simulink model "machine_model_A_test"  (R2018b)
settings: Solver=ode45  StartTime=0.0  StopTime=65  RelTol=1e-3
PreLoadFcn:
  | load_system('../simulink_reference_models/test_sequence_lib');
InitFcn:
  | close all
  | clear all
  | 
  | T_CNTL = 1/5e3;
  | 
  | P_NOM = 1e6;
  | VLL_NOM = 480;
  | F_NOM = 60;
  | W_NOM = 2 * 3.14159265 * F_NOM;
  | 
  | Z_BASE = VLL_NOM * VLL_NOM / P_NOM;
  | L_BASE = Z_BASE / W_NOM;
  | C_BASE = 1 / (W_NOM * Z_BASE);
libraries: simulink x4, test_sequence_lib x4
settings Model: SimulationMode=rapid-accelerator  Creator=HussamAlatrash  LastModifiedBy=ahhei
settings DataIOCC: ReturnWorkspaceOutputs=on
settings DebuggingCC: UnconnectedInputMsg=none  UnconnectedOutputMsg=none  UnconnectedLineMsg=none
settings ModelReferenceCC: EnableRefExpFcnMdlSchedulingChecks=off
settings RTWCC: Description=Generic Real-Time Target
settings ConfigComp: CovBoundaryAbsTol=1.0e-5

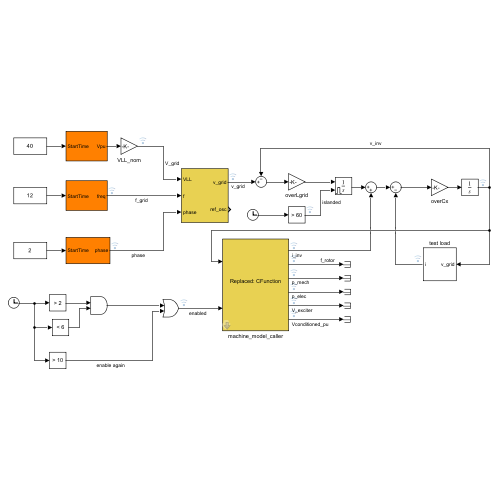
[thumbnail: Simulink's stored preview of the top-level diagram]
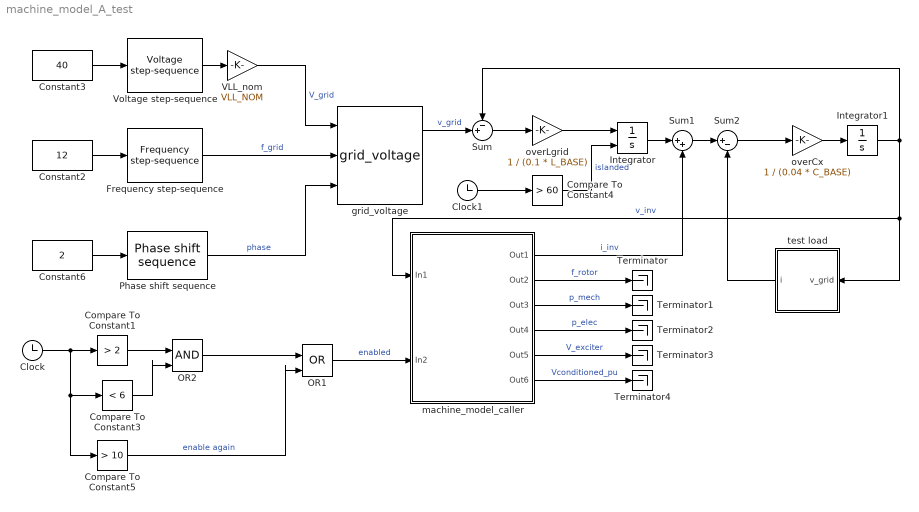
== system machine_model_A_test ==
  Clock : Clock
  Clock1 : Clock
  Compare To Constant1 : simulink/Logic and Bit Operations/Compare To Constant  relop=>  const=2  OutDataTypeStr=boolean
  Compare To Constant3 : simulink/Logic and Bit Operations/Compare To Constant  relop=<  const=6  OutDataTypeStr=boolean
  Compare To Constant4 : simulink/Logic and Bit Operations/Compare To Constant  relop=>  const=60  OutDataTypeStr=boolean
  Compare To Constant5 : simulink/Logic and Bit Operations/Compare To Constant  relop=>  const=10  OutDataTypeStr=boolean
  Constant2 : Constant  Value=12
  Constant3 : Constant  Value=40
  Constant6 : Constant  Value=2
  Frequency step-sequence : test_sequence_lib/Frequency step-sequence  SystemSampleTime=-1  EmptyChoice=off  PassThrough=off  PassThroughVariantControl=(default)  EmptyChoiceVariantControl=(default)  Latency=0  AutoFrameSizeCalculation=off
  Integrator : Integrator  ExternalReset=level
  Integrator1 : Integrator
  OR1 : Logic  Operator=OR  IconShape=distinctive  AllPortsSameDT=off  OutDataTypeStr=boolean
  OR2 : Logic  IconShape=distinctive  AllPortsSameDT=off  OutDataTypeStr=boolean
  Phase shift sequence : test_sequence_lib/Phase shift sequence  SystemSampleTime=-1  EmptyChoice=off  PassThrough=off  PassThroughVariantControl=(default)  EmptyChoiceVariantControl=(default)  Latency=0  AutoFrameSizeCalculation=off
  Sum : Sum  Inputs=-+|
  Sum1 : Sum  Inputs=|++
  Sum2 : Sum  Inputs=|+-
  Terminator{,1..4} (5 alike) : Terminator
  VLL_nom : Gain  Gain=VLL_NOM
  Voltage step-sequence : test_sequence_lib/Voltage step-sequence  SystemSampleTime=-1  EmptyChoice=off  PassThrough=off  PassThroughVariantControl=(default)  EmptyChoiceVariantControl=(default)  Latency=0  AutoFrameSizeCalculation=off
  grid_voltage : test_sequence_lib/grid_voltage  SystemSampleTime=-1  EmptyChoice=off  PassThrough=off  PassThroughVariantControl=(default)  EmptyChoiceVariantControl=(default)  Latency=0  AutoFrameSizeCalculation=off
  machine_model_caller : Subsystem  Description=Replaced Block  mask(Replaced Block){}
      mask help: This block has been replaced with an empty subsystem because it used functionality that is unavailable in Simulink R2018b.
      mask Display: fprintf('Replaced: %s\n','CFunction')
  overCx : Gain  Gain=1 / (0.04 * C_BASE)
  overLgrid : Gain  Gain=1 / (0.1 * L_BASE)
  test load : Subsystem
  wires:
  Constant2/1 -> Frequency step-sequence/1
  Constant3/1 -> Voltage step-sequence/1
  grid_voltage/1 -> Sum/2  "v_grid"
  test load/1(i) -> Sum2/2
  Frequency step-sequence/1 -> grid_voltage/2  "f_grid"
  Constant6/1 -> Phase shift sequence/1
  Voltage step-sequence/1 -> VLL_nom/1
  VLL_nom/1 -> grid_voltage/1  "V_grid"
  Phase shift sequence/1 -> grid_voltage/3  "phase"
  machine_model_caller/2(Out2) -> Terminator/1  "f_rotor"
  overLgrid/1 -> Integrator/1
  Integrator/1 -> Sum1/1
  Integrator1/1 -> test load/1(v_grid), machine_model_caller/1(In1), Sum/1  "v_inv"
  overCx/1 -> Integrator1/1
  Sum2/1 -> overCx/1
  Sum1/1 -> Sum2/1
  Sum/1 -> overLgrid/1
  machine_model_caller/1(Out1) -> Sum1/2  "i_inv"
  machine_model_caller/3(Out3) -> Terminator1/1  "p_mech"
  machine_model_caller/4(Out4) -> Terminator2/1  "p_elec"
  machine_model_caller/5(Out5) -> Terminator3/1  "V_exciter"
  machine_model_caller/6(Out6) -> Terminator4/1  "Vconditioned_pu"
  Clock/1 -> Compare To Constant3/1, Compare To Constant5/1, Compare To Constant1/1
  Compare To Constant1/1 -> OR2/1
  Clock1/1 -> Compare To Constant4/1
  Compare To Constant4/1 -> Integrator/2  "islanded"
  Compare To Constant3/1 -> OR2/2
  OR2/1 -> OR1/1
  Compare To Constant5/1 -> OR1/2  "enable again"
  OR1/1 -> machine_model_caller/2(In2)  "enabled"

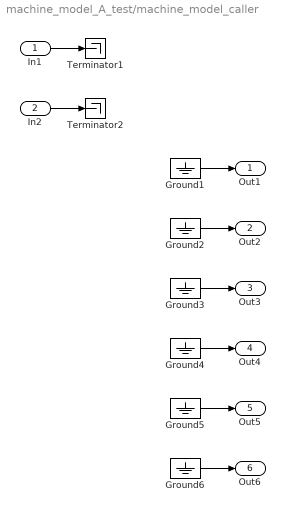
== system machine_model_A_test/machine_model_caller ==
  In1 : Inport
  In2 : Inport  Port=2
  Ground{1..6} (6 alike) : Ground
  Terminator1 : Terminator
  Terminator2 : Terminator
  Out1 : Outport
  Out2 : Outport  Port=2
  Out3 : Outport  Port=3
  Out4 : Outport  Port=4
  Out5 : Outport  Port=5
  Out6 : Outport  Port=6
  wires:
  Ground6/1 -> Out6/1
  Ground5/1 -> Out5/1
  Ground4/1 -> Out4/1
  Ground3/1 -> Out3/1
  Ground2/1 -> Out2/1
  Ground1/1 -> Out1/1
  In2/1 -> Terminator2/1
  In1/1 -> Terminator1/1

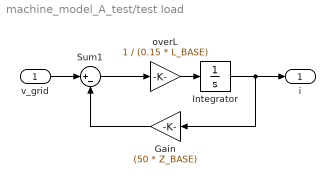
== system machine_model_A_test/test load ==
  v_grid : Inport
  Gain : Gain  Gain=(50 * Z_BASE)
  Integrator : Integrator
  Sum1 : Sum  Inputs=|+-
  overL : Gain  Gain=1 / (0.15 * L_BASE)
  i : Outport
  wires:
  v_grid/1 -> Sum1/1
  overL/1 -> Integrator/1
  Sum1/1 -> overL/1
  Integrator/1 -> i/1, Gain/1
  Gain/1 -> Sum1/2
